simulink model "dc_motor_pd_encoder"  (R2024b)
settings: Solver=VariableStepAuto  StartTime=0.0  StopTime=3  RelTol=1e-3
settings Model: Creator=Grishma  LastModifiedBy=Grishma

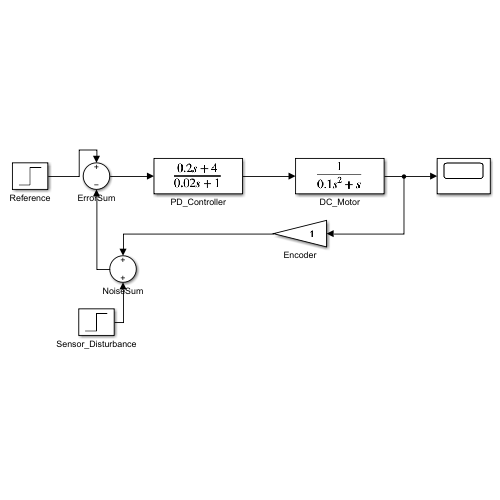
[thumbnail: Simulink's stored preview of the top-level diagram]
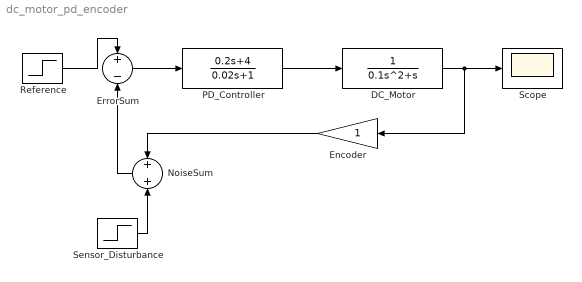
== system dc_motor_pd_encoder ==
  DC_Motor : TransferFcn  Denominator=[0.1 1 0]
  Encoder : Gain
  ErrorSum : Sum  Inputs=+-
  NoiseSum : Sum
  PD_Controller : TransferFcn  Numerator=[0.2 4]  Denominator=[0.02 1]
  Reference : Step  Time=0  SampleTime=0
  Scope : Scope
  Sensor_Disturbance : Step  After=0.05  SampleTime=0
  wires:
  Reference/1 -> ErrorSum/1
  NoiseSum/1 -> ErrorSum/2
  ErrorSum/1 -> PD_Controller/1
  PD_Controller/1 -> DC_Motor/1
  DC_Motor/1 -> Scope/1, Encoder/1
  Encoder/1 -> NoiseSum/1
  Sensor_Disturbance/1 -> NoiseSum/2
